simulink model "UAM_Hexa_PD_Diff_Pos_Man_PX4"  (R2026a)
settings: Solver=ode4  StopTime=tf  FixedStep=0.01
values from neighbouring files (symbols this model uses):
  ArmConstants = struct('l1_dim', l1_dim,                        'l2_dim', l2_dim,                        'Hexa_to_joint_L', L,                        'Mass1', ml1,                        'Mass2', ml2,                        'Inertia1', Hl1,                        'Inertia2', Hl2,                        'MC1', c1,                        'MC2', c2,                        'Servos', Servos)    [init_model.m]    (also in init_var.m)
  Differentiator = struct('G1', G1 ,     'G2', G2 ,     'Q1', Q1 ,     'Q2', Q2 ,     'w1', w1 ,     'w2', w2 ,     'p1', p1 ,     'p2', p2)    [init_model.m]    (also in init_var.m)
  HexaConstants = struct('Mass', mb,                         'Inertia', J ,                         'allo', allo,                          'invallo', invallo,                         'kT', kT)    [init_model.m]    (also in init_var.m)
libraries: simulink x2
settings Model: Creator=Carlos Fabian  LastModifiedBy=Carlos Fabian
settings ExplorerConfigSet: InternalSimMechanicsExplorerSettings=|
  | <ExplorerConfiguration>
  | 
  |   <canonicalview>default</canonicalview>
  | 
  |   <TilePanel>
  |     <TileInfo>
  |       <Tiles Columns="1" Count="1" Height="513" Rows="1" Width="1199">
  |         <Row Weight="1"/>
  |         <Column Weight="1"/>
  |         <Tile Height="1" Width="1" X="0" Y="0"/>
  |       </Tiles>
  |     </TileInfo>
  |     <SceneInfo>
  |       <SceneViewer>
  |         <IsThisViewStd>
  |           <IsStandardView>off</IsStandardView>
  |           <StandardViewName>Front</StandardViewName>
  |         </IsThisViewStd>
  |         <BGColor>
  |           <R>1</R>
  |           <G>1</G>
  |           <B>1</B>
  |           <A>1</A>
  |         </BGColor>
  |         <Camera>
  |           <DoPerspective>off</DoPerspective>
  |           <Position>
  |             <X>16.563809413425133</X>
  |             <Y>-16.563809413425133</Y>
  |             <Z>17.346953838391503</Z>
  |           </Position>
  |           <Center>
  |             <X>0</X>
  |             <Y>0</Y>
  |             <Z>0.78314442496637693</Z>
  |           </Center>
  |           <Up>
  |             <X>-0.40824829046386285</X>
  |             <Y>0.40824829046386285</Y>
  |             <Z>0.81649658092772603</Z>
  |           </Up>
  |           <XLim>3.39184009237395</XLim>
  |           <YLim>3.39184009237395</YLim>
  |           <ViewLimDist>0.01</ViewLimDist>
  |         </Camera>
  |       </SceneViewer>
  |     </SceneInfo>
  |   </TilePanel>
  | 
  |   <MechEditorPanel>
  |     <GfxPanelCameraMap/>
  |     <Cameras/>
  |     <VideoCreator>
  |       <IncludeTiles>All</IncludeTiles>
  |       <IncludeTime>on</IncludeTime>
  |       <IncludeWorldFrame>off</IncludeWorldFrame>
  |       <PlaybackSpeedRatio>8</PlaybackSpeedRatio>
  |       <FrameRate>24</FrameRate>
  |       <FrameSize>auto</FrameSize>
  |       <VideoFormat>MotionJPEGAVI</VideoFormat>
  |     </VideoCreator>
  |   </MechEditorPanel>
  | 
  |   <PlaybackSettings>
  |     <PlaybackSpeedFactor>4</PlaybackSpeedFactor>
  |   </PlaybackSettings>
  | 
  | </ExplorerConfiguration>

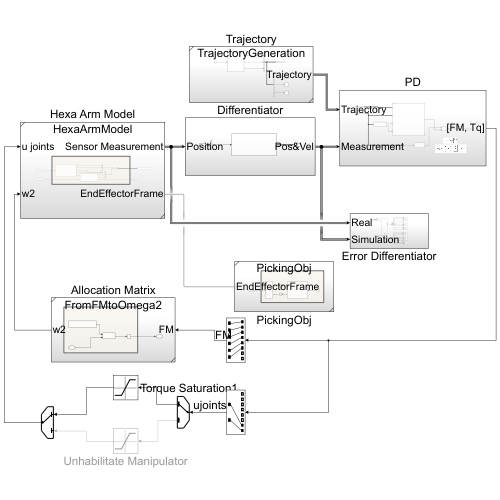
[thumbnail: Simulink's stored preview of the top-level diagram]
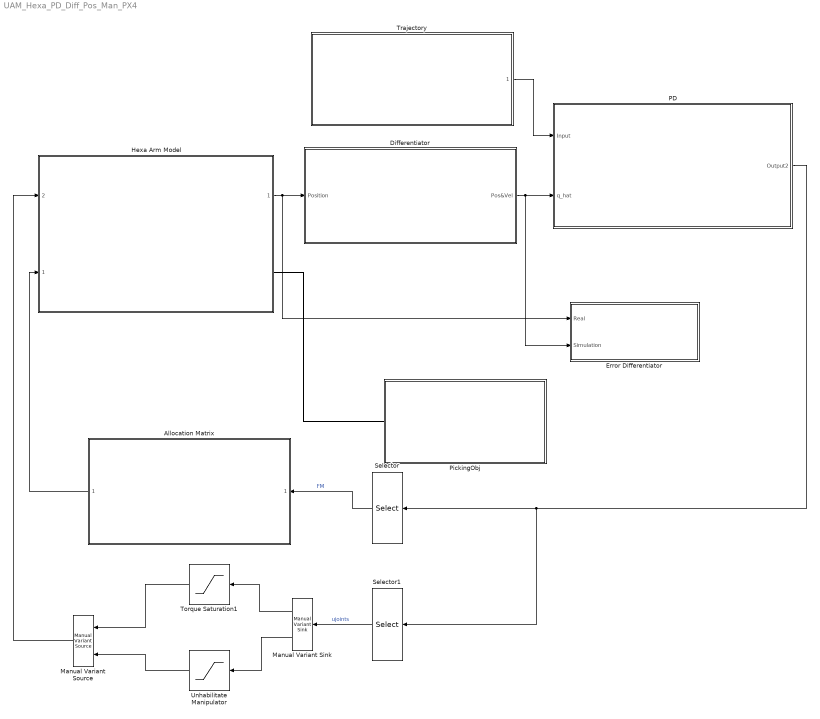
== system UAM_Hexa_PD_Diff_Pos_Man_PX4 ==
  Allocation Matrix : Subsystem  ReferencedSubsystem=FromFMtoOmega2
  Differentiator : Subsystem
  Error Differentiator : Subsystem
  Hexa Arm Model : Subsystem  ReferencedSubsystem=HexaArmModel
      settings: PortSchema="{\"entries\":[{\"content\":{\"sides\":[{\"content\":{\"connectorIds\":[\"In2\",\"In1\"]},\"type\":\"ConnectorPlacement.EquallySpacedRectSide\",\"uuid\":\"8c321911-c61a-4c60-b031-eeaf4c8b5083\"},{\"content\":{\"connectorIds\":[\"Out1\",\"RConn1\"],\"side\":\"RIGHT\"},\"type\":\"ConnectorPlacement.EquallySpacedRectSide\",\"uuid\":\"3ad1588f-e2f8-4666-8b86-318f5207193d\"},{\"content\":{\"side\":\"TOP\"},\"type\":\"ConnectorPlacement.EquallySpacedRectSide\",\"uuid\":\"710cc49c-59c4-4f69-a558-4588d1d119c0\"}]},\"type\":\"ConnectorPlacement.EquallySpacedConnector\",\"uuid\":\"3e8cca1f-f7f1-4f31-9eba-ef93ff8e81e8\"}],\"packageUris\":[\"http://schema.mathworks.com/mf0/Connector/R2020b\"],\"version\":\"1.0\"}"
  Manual Variant Sink : simulink/Signal Routing/Manual Variant Sink  NumChoices=2  LabelModeActiveChoice=V_1
  Manual Variant Source : simulink/Signal Routing/Manual Variant Source  NumChoices=2  LabelModeActiveChoice=V_1
  PD : Subsystem
  PickingObj : Subsystem  ReferencedSubsystem=PickingObj
  Selector : Selector  InputPortWidth=8  IndexOptions=Index vector (dialog)  Indices=1:6  OutputSizes=1
  Selector1 : Selector  InputPortWidth=8  IndexOptions=Index vector (dialog)  Indices=7:8  OutputSizes=1
  Torque Saturation1 : Saturate  UpperLimit=ArmConstants.Servos.T1max  LowerLimit=-ArmConstants.Servos.T1max
  Trajectory : Subsystem  ReferencedSubsystem=TrajectoryGeneration
  Unhabilitate Manipulator : Saturate  UpperLimit=ArmConstants.Servos.T1max-2.4999999999  LowerLimit=-ArmConstants.Servos.T1max+2.4999999999
  wires:
  Selector/1 -> Allocation Matrix/1  "FM"
  PD/1(Output2) -> Selector/1, Selector1/1
  Manual Variant Source/1 -> Hexa Arm Model/2
  Selector1/1 -> Manual Variant Sink/1  "ujoints"
  Trajectory/1 -> PD/1(Input)
  Allocation Matrix/1 -> Hexa Arm Model/1
  Hexa Arm Model/1 -> Error Differentiator/1(Real), Differentiator/1(Position)
  Differentiator/1(Pos&Vel) -> Error Differentiator/2(Simulation), PD/2(q_hat)
  Manual Variant Sink/1 -> Torque Saturation1/1
  Manual Variant Sink/2 -> Unhabilitate Manipulator/1
  Torque Saturation1/1 -> Manual Variant Source/1
  Unhabilitate Manipulator/1 -> Manual Variant Source/2
  connections:
  Hexa Arm Model/RConn1 -- PickingObj/LConn1

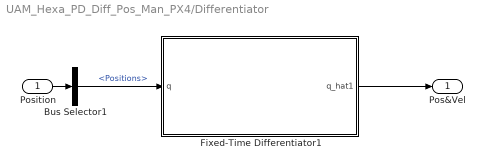
== system UAM_Hexa_PD_Diff_Pos_Man_PX4/Differentiator ==
  Position : Inport
  Bus Selector1 : BusSelector  OutputSignals=Positions
  Fixed-Time Differentiator1 : Subsystem
      settings: PortSchema="{\"entries\":[{\"content\":{\"sides\":[{\"content\":{\"connectorIds\":[\"Out1\"]},\"type\":\"ConnectorPlacement.EquallySpacedRectSide\",\"uuid\":\"d79ec49c-5563-41e0-ac59-6e897bc19fda\"},{\"content\":{\"connectorIds\":[\"In1\"],\"side\":\"RIGHT\"},\"type\":\"ConnectorPlacement.EquallySpacedRectSide\",\"uuid\":\"1255043e-c90e-4bae-9fb4-4fa06f36f53e\"},{\"content\":{\"side\":\"TOP\"},\"type\":\"ConnectorPlacement.EquallySpacedRectSide\",\"uuid\":\"823ada36-3f22-4ee3-87a1-180276f622bc\"}]},\"type\":\"ConnectorPlacement.EquallySpacedConnector\",\"uuid\":\"7403b609-b333-4977-a854-ed7a71f74338\"}],\"packageUris\":[\"http://schema.mathworks.com/mf0/Connector/R2020b\"],\"version\":\"1.0\"}"
  Pos&Vel : Outport
  wires:
  Bus Selector1/1 -> Fixed-Time Differentiator1/1(q)  "<Positions>"
  Position/1 -> Bus Selector1/1
  Fixed-Time Differentiator1/1(q_hat1) -> Pos&Vel/1

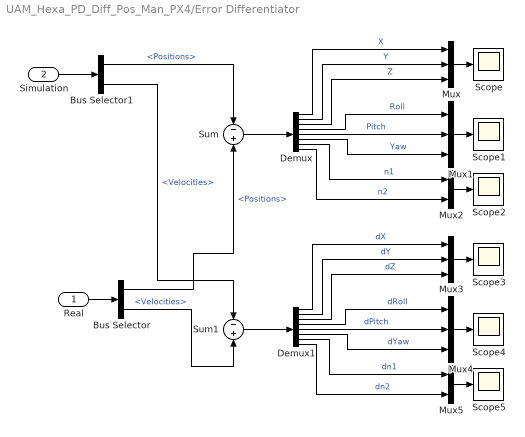
== system UAM_Hexa_PD_Diff_Pos_Man_PX4/Error Differentiator ==
  Real : Inport
  Simulation : Inport  Port=2
  Bus Selector : BusSelector  OutputSignals=Positions,Velocities
  Bus Selector1 : BusSelector  OutputSignals=Positions,Velocities
  Demux : Demux  Outputs=8
  Demux1 : Demux  Outputs=8
  Mux{,1,3..4} (4 alike) : Mux  Inputs=3
  Mux2 : Mux  Inputs=2
  Mux5 : Mux  Inputs=2
  Scope{,1..5} (6 alike) : Scope
      Scope settings: ActiveDisplayYMinimum=-0.11516314203526654  ActiveDisplayYMaximum=0.12253392651728615
      Scope1 settings: ActiveDisplayYMinimum=-0.039456080037096539  ActiveDisplayYMaximum=0.028206770020752458  DataLoggingVariableName=ScopeData4
      Scope2 settings: ActiveDisplayYMinimum=-0.097057334019579361  ActiveDisplayYMaximum=0.091379254090405648  DataLoggingVariableName=ScopeData5
      Scope3 settings: ActiveDisplayYMinimum=-0.12118491948489385  ActiveDisplayYMaximum=0.25198076657940688  DataLoggingVariableName=ScopeData6
      Scope4 settings: ActiveDisplayYMinimum=-0.049702476607807689  ActiveDisplayYMaximum=0.057495988286683834  DataLoggingVariableName=ScopeData7
      Scope5 settings: ActiveDisplayYMinimum=-11.414042765802602  ActiveDisplayYMaximum=7.1811721637788093  DataLoggingVariableName=ScopeData8
  Sum : Sum  Inputs=-+
  Sum1 : Sum  Inputs=-+
  wires:
  Mux2/1 -> Scope2/1
  Sum/1 -> Demux/1
  Mux1/1 -> Scope1/1
  Bus Selector1/1 -> Sum/1  "<Positions>"
  Demux/8 -> Mux2/2  "n2"
  Bus Selector/2 -> Sum1/2  "<Velocities>"
  Demux/7 -> Mux2/1  "n1"
  Mux/1 -> Scope/1
  Demux/1 -> Mux/1  "X"
  Demux/4 -> Mux1/1  "Roll"
  Demux/6 -> Mux1/3  "Yaw"
  Demux/5 -> Mux1/2  "Pitch"
  Demux/3 -> Mux/3  "Z"
  Bus Selector/1 -> Sum/2  "<Positions>"
  Demux/2 -> Mux/2  "Y"
  Bus Selector1/2 -> Sum1/1  "<Velocities>"
  Simulation/1 -> Bus Selector1/1
  Real/1 -> Bus Selector/1
  Demux1/8 -> Mux5/2  "dn2"
  Mux4/1 -> Scope4/1
  Sum1/1 -> Demux1/1
  Mux5/1 -> Scope5/1
  Demux1/4 -> Mux4/1  "dRoll"
  Demux1/6 -> Mux4/3  "dYaw"
  Demux1/2 -> Mux3/2  "dY"
  Demux1/1 -> Mux3/1  "dX"
  Mux3/1 -> Scope3/1
  Demux1/5 -> Mux4/2  "dPitch"
  Demux1/7 -> Mux5/1  "dn1"
  Demux1/3 -> Mux3/3  "dZ"

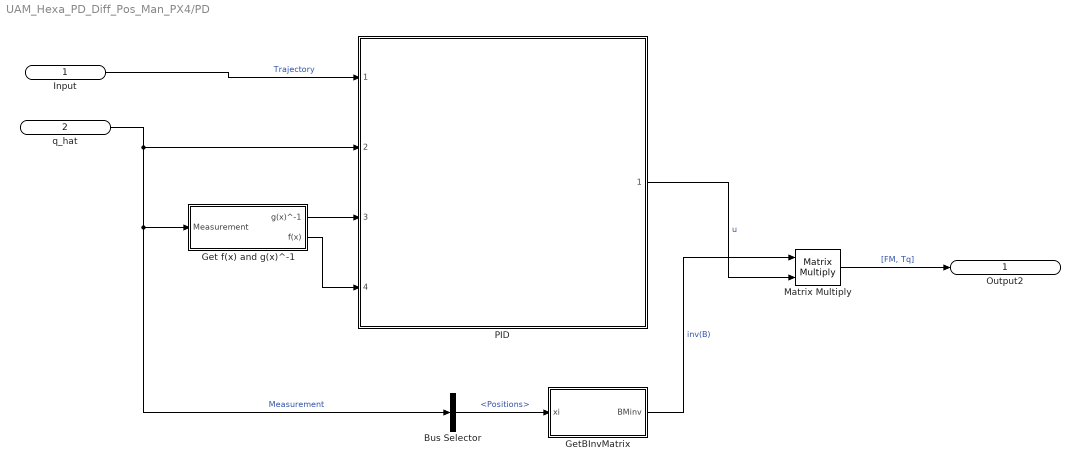
== system UAM_Hexa_PD_Diff_Pos_Man_PX4/PD ==
  Input : Inport
  q_hat : Inport  Port=2
  Bus Selector : BusSelector  OutputSignals=Positions
  Get f(x) and g(x)^-1 : Subsystem
  GetBInvMatrix : MATLAB Function  TreatAsAtomicUnit=on
  Matrix Multiply : Product  Multiplication=Matrix(*)
  PID : Subsystem  ReferencedSubsystem=PIDController
  Output2 : Outport
  wires:
  q_hat/1 -> Get f(x) and g(x)^-1/1(Measurement), Bus Selector/1, PID/2  "Measurement"
  Input/1 -> PID/1  "Trajectory"
  Bus Selector/1 -> GetBInvMatrix/1(xi)  "<Positions>"
  GetBInvMatrix/1(BMinv) -> Matrix Multiply/1  "inv(B)"
  PID/1 -> Matrix Multiply/2  "u"
  Matrix Multiply/1 -> Output2/1  "[FM, Tq]"
  Get f(x) and g(x)^-1/1(g(x)^-1) -> PID/3
  Get f(x) and g(x)^-1/2(f(x)) -> PID/4

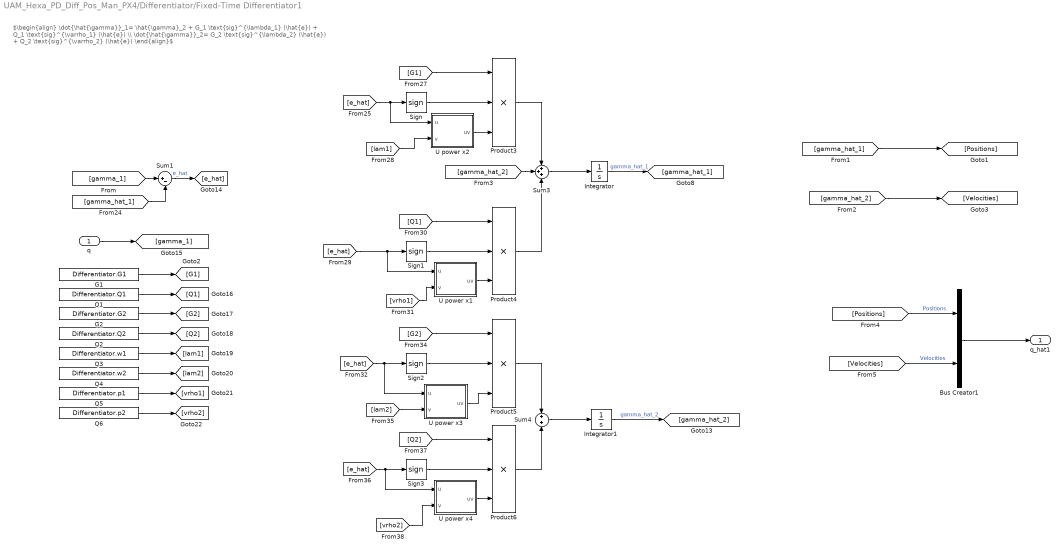
== system UAM_Hexa_PD_Diff_Pos_Man_PX4/Differentiator/Fixed-Time Differentiator1 ==
  note: $\begin{align} \dot{\hat{\gamma}}_1= \hat{\gamma}_2 + G_1 \text{sig}^{\lambda_1} (\hat{e}) + Q_1 \text{sig}^{\varrho_1} (\hat{e}) \\ \dot{\hat{\gamma}}_2= G_2 \text{sig}^{\lambda_2} (\hat{e}) + Q_2 \text{sig}^{\varrho_2} (\hat{e}) \end{align}$
  q : Inport
  Bus Creator1 : BusCreator  Inputs=2
  G1 : Constant  Value=Differentiator.G1
  G2 : Constant  Value=Differentiator.G2
  Integrator : Integrator  InitialCondition=[0; 0; 0.28; 0; 0; 0; 0; 0]  IgnoreLimit=on
  Integrator1 : Integrator  InitialCondition=[0; 0; 0; 0; 0; 0; 0; 0]  IgnoreLimit=on
  Product{3..6} (4 alike) : Product  Inputs=3
  Q1 : Constant  Value=Differentiator.Q1
  Q2 : Constant  Value=Differentiator.Q2
  Q3 : Constant  Value=Differentiator.w1
  Q4 : Constant  Value=Differentiator.w2
  Q5 : Constant  Value=Differentiator.p1
  Q6 : Constant  Value=Differentiator.p2
  Sign{,1..3} (4 alike) : Signum
  Sum1 : Sum  Inputs=|+-
  Sum3 : Sum  Inputs=+++
  Sum4 : Sum  Inputs=+|+
  U power x1 : MATLAB Function  TreatAsAtomicUnit=on
  U power x2 : MATLAB Function  TreatAsAtomicUnit=on
  U power x3 : MATLAB Function  TreatAsAtomicUnit=on
  U power x4 : MATLAB Function  TreatAsAtomicUnit=on
  q_hat1 : Outport
  wires:
  Product6/1 -> Sum4/2
  G1/1 -> [G1]
  Sum1/1 -> [e_hat]  "e_hat"
  Sign3/1 -> Product6/2
  [gamma_hat_1] -> Sum1/2
  Q5/1 -> [vrho1]
  Q1/1 -> [Q1]
  Q6/1 -> [vrho2]
  [vrho2] -> U power x4/2(v)
  Q2/1 -> [Q2]
  [G1] -> Product3/1
  G2/1 -> [G2]
  Sign2/1 -> Product5/2
  Q4/1 -> [lam2]
  Product5/1 -> Sum4/1
  [gamma_1] -> Sum1/1
  [lam2] -> U power x3/2(v)
  [G2] -> Product5/1
  [Q2] -> Product6/1
  Product3/1 -> Sum3/1
  Sign/1 -> Product3/2
  Q3/1 -> [lam1]
  q/1 -> [gamma_1]
  Integrator/1 -> [gamma_hat_1]  "gamma_hat_1"
  [gamma_hat_2] -> [Velocities]
  Sum4/1 -> Integrator1/1
  Sum3/1 -> Integrator/1
  [gamma_hat_2] -> Sum3/2
  Product4/1 -> Sum3/3
  Sign1/1 -> Product4/2
  [vrho1] -> U power x1/2(v)
  [Q1] -> Product4/1
  [e_hat] -> U power x1/1(u), Sign1/1
  [e_hat] -> U power x3/1(u), Sign2/1
  [e_hat] -> U power x4/1(u), Sign3/1
  [e_hat] -> U power x2/1(u), Sign/1
  U power x2/1(uv) -> Product3/3
  [lam1] -> U power x2/2(v)
  U power x1/1(uv) -> Product4/3
  U power x3/1(uv) -> Product5/3
  U power x4/1(uv) -> Product6/3
  [gamma_hat_1] -> [Positions]
  Bus Creator1/1 -> q_hat1/1
  [Positions] -> Bus Creator1/1  "Positions"
  [Velocities] -> Bus Creator1/2  "Velocities"
  Integrator1/1 -> [gamma_hat_2]  "gamma_hat_2"

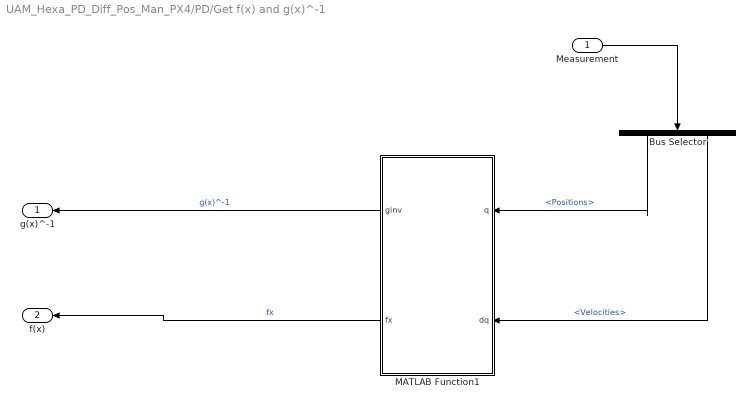
== system UAM_Hexa_PD_Diff_Pos_Man_PX4/PD/Get f(x) and g(x)^-1 ==
  Measurement : Inport
  Bus Selector : BusSelector  OutputSignals=Positions,Velocities
  MATLAB Function1 : MATLAB Function  TreatAsAtomicUnit=on
  g(x)^-1 : Outport
  f(x) : Outport  Port=2
  wires:
  MATLAB Function1/2(fx) -> f(x)/1  "fx"
  MATLAB Function1/1(ginv) -> g(x)^-1/1  "g(x)^-1"
  Measurement/1 -> Bus Selector/1
  Bus Selector/1 -> MATLAB Function1/1(q)  "<Positions>"
  Bus Selector/2 -> MATLAB Function1/2(dq)  "<Velocities>"

== matlab function UAM_Hexa_PD_Diff_Pos_Man_PX4/PD/GetBInvMatrix ==
  data: xi input; BMinv output
function BMinv = GetBInvMatrix(xi)

% phi = xi(4);
% th  = xi(5);
% psi = xi(6);
% 
% BM1=[cos(phi)*cos(th),-cos(phi)*sin(psi)+cos(psi)*sin(phi)*sin(th), ...
%     sin(phi)*sin(psi)+cos(phi)*cos(psi)*sin(th),0,0,0;...
%     cos(th)*sin(psi), cos(phi)*cos(psi)+sin(phi)*sin(psi)*sin(th),...
%     -cos(psi)*sin(phi)+cos(phi)*sin(psi)*sin(phi),0,0,0;...
%     -sin(th),cos(th)*sin(psi),cos(phi)*cos(th),0,0,0;...
%     0,0,0,1,sin(phi)*tan(th),cos(phi)*tan(th);...
%     0,0,0,0,cos(phi),-sin(phi);0,0,0,0,sec(th)*sin(phi),cos(phi)*sec(th)];

BM1 = BMatrix(xi);

BM = blkdiag(BM1, eye(2,2));

BMinv = inv(BM);

end

== matlab function UAM_Hexa_PD_Diff_Pos_Man_PX4/Differentiator/Fixed-Time Differentiator1/U power x2 ==
  data: u input; uv output; v input
function uv = u_x(u, v)
i = 1;
uv = zeros(8,1);
for i=1:8
    absolute = abs(u(i));
    uv(i) = absolute ^ v(i);
    % if absolute < 0.00005
    %     uv(i) = 0;
    % else
    %     uv(i) = absolute ^ v(i);
    % end
end
end

== matlab function UAM_Hexa_PD_Diff_Pos_Man_PX4/Differentiator/Fixed-Time Differentiator1/U power x1 ==
  data: u input; uv output; v input
function uv = u_x(u, v)
i = 1;
uv = zeros(8,1);
for i=1:8
    absolute = abs(u(i));
    uv(i) = absolute ^ v(i);
    % if absolute < 0.00005
    %     uv(i) = 0;
    % else
    %     uv(i) = absolute ^ v(i);
    % end
end
end

== matlab function UAM_Hexa_PD_Diff_Pos_Man_PX4/Differentiator/Fixed-Time Differentiator1/U power x3 ==
  data: u input; uv output; v input
function uv = u_x(u, v)
i = 1;
uv = zeros(8,1);
for i=1:8
    absolute = abs(u(i));
    uv(i) = absolute ^ v(i);
    % if absolute < 0.00005
    %     uv(i) = 0;
    % else
    %     uv(i) = absolute ^ v(i);
    % end
end
end

== matlab function UAM_Hexa_PD_Diff_Pos_Man_PX4/Differentiator/Fixed-Time Differentiator1/U power x4 ==
  data: u input; uv output; v input
function uv = u_x(u, v)
i = 1;
uv = zeros(8,1);
for i=1:8
    absolute = abs(u(i));
    uv(i) = absolute ^ v(i);
    % if absolute < 0.00005
    %     uv(i) = 0;
    % else
    %     uv(i) = absolute ^ v(i);
    % end
end
end

== matlab function UAM_Hexa_PD_Diff_Pos_Man_PX4/PD/Get f(x) and g(x)^-1/MATLAB Function1 ==
  data: q input; dq input; HexaConstants parameter; ginv output; fx output; ArmConstants parameter
function [ginv, fx] = Get_DCG_Hexa(q, dq, HexaConstants, ArmConstants)

DM = DMatrix(q, HexaConstants, ArmConstants);
CM = CMatrix(q, dq, HexaConstants, ArmConstants);
Gv = GVector(q, HexaConstants, ArmConstants);

ginv = DM;

fx = DM\( -CM*dq - Gv );

end
